simulink subsystem "FlexibleDriveline"  (R2025b)
settings: Solver=VariableStepAuto  StartTime=0.0  StopTime=10.0  RelTol=1e-3
PreLoadFcn:
  | FlexibleDrivelineParams;
undefined symbols (not defined in the file or in its folder): flexDLParams, fs
libraries: fl_lib x41, sdl_lib x24, nesl_utility x3
(part 1 of 2)
settings Model: Creator=shachind  LastModifiedBy=shachind

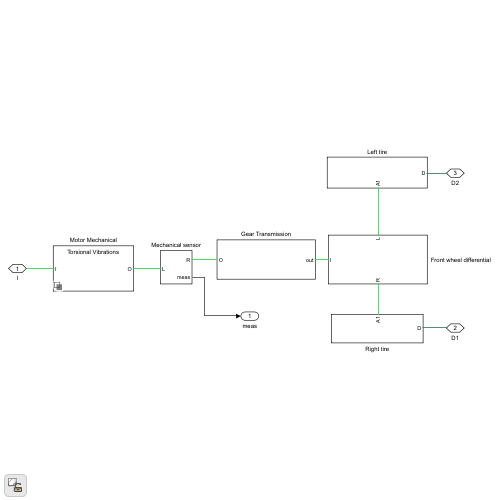
[thumbnail: Simulink's stored preview of the top-level diagram]
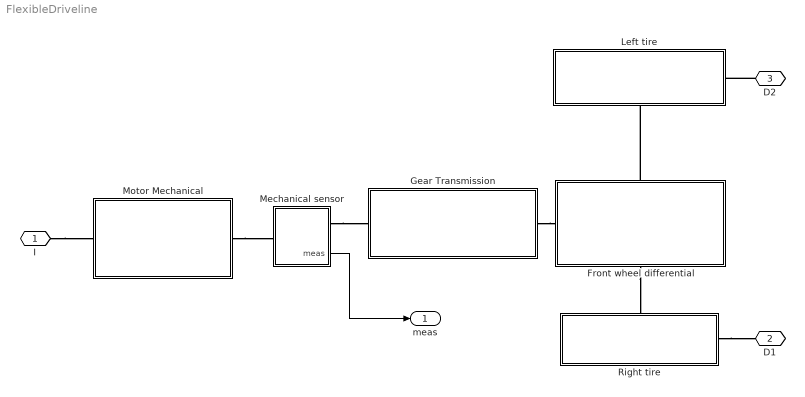
== system FlexibleDriveline ==
  Front wheel differential : Subsystem
      settings: PortSchema="{\"entries\":[{\"content\":{\"sides\":[{\"content\":{\"connectorIds\":[\"LConn1\"]},\"type\":\"ConnectorPlacement.EquallySpacedRectSide\",\"uuid\":\"c11434d0-9930-428a-bdcc-d2cb24030201\"},{\"content\":{\"connectorIds\":[\"RConn1\"],\"side\":\"RIGHT\"},\"type\":\"ConnectorPlacement.EquallySpacedRectSide\",\"uuid\":\"94e78a84-1cc1-4194-8e32-79b35f643a00\"},{\"content\":{\"side\":\"TOP\"},\"type\":\"ConnectorPlacement.EquallySpacedRectSide\",\"uuid\":\"2a2ff05c-1e68-4433-96e8-1c1d7698d135\"},{\"content\":{\"connectorIds\":[\"RConn2\"],\"side\":\"BOTTOM\"},\"type\":\"ConnectorPlacement.EquallySpacedRectSide\",\"uuid\":\"79f74731-f04d-4ec7-8450-045a74f69ecc\"}]},\"type\":\"ConnectorPlacement.EquallySpacedConnector\",\"uuid\":\"ade08aca-446e-4c23-b476-7b46661d2103\"}],\"packageUris\":[\"http://schema.mathworks.com/mf0/Connector/R2020b\"],\"version\":\"1.0\"}"
  Gear Transmission : Subsystem
  Left tire : Subsystem
      settings: PortSchema="{\"entries\":[{\"content\":{\"sides\":[{\"content\":{},\"type\":\"ConnectorPlacement.EquallySpacedRectSide\",\"uuid\":\"a6e63744-e74e-4c59-9a73-9f5bb4c6dc5e\"},{\"content\":{\"connectorIds\":[\"RConn1\"],\"side\":\"RIGHT\"},\"type\":\"ConnectorPlacement.EquallySpacedRectSide\",\"uuid\":\"cd80d7a6-bc64-46ff-87eb-327b10d625d4\"},{\"content\":{\"side\":\"TOP\"},\"type\":\"ConnectorPlacement.EquallySpacedRectSide\",\"uuid\":\"654a6e45-7395-4805-a08f-34f7a106fd1a\"},{\"content\":{\"connectorIds\":[\"RConn2\"],\"side\":\"BOTTOM\"},\"type\":\"ConnectorPlacement.EquallySpacedRectSide\",\"uuid\":\"572e738d-5229-4313-b0e3-7599b587bb85\"}]},\"type\":\"ConnectorPlacement.EquallySpacedConnector\",\"uuid\":\"3d8eeb69-cd59-4894-aa80-d96e9faae830\"}],\"packageUris\":[\"http://schema.mathworks.com/mf0/Connector/R2020b\"],\"version\":\"1.0\"}"
  Mechanical sensor : Subsystem
      settings: PortSchema="{\"entries\":[{\"content\":{\"sides\":[{\"content\":{\"connectorIds\":[\"LConn1\",\"Out1\"]},\"type\":\"ConnectorPlacement.EquallySpacedRectSide\",\"uuid\":\"9d0b7eaf-5dbc-4711-a9f9-5254d5ad2438\"},{\"content\":{\"connectorIds\":[\"RConn1\"],\"side\":\"RIGHT\"},\"type\":\"ConnectorPlacement.EquallySpacedRectSide\",\"uuid\":\"1084bd7e-accf-404d-815d-6b48331d5fd1\"},{\"content\":{\"side\":\"TOP\"},\"type\":\"ConnectorPlacement.EquallySpacedRectSide\",\"uuid\":\"4e1c109f-5704-45c2-8a88-7bde344122da\"}]},\"type\":\"ConnectorPlacement.EquallySpacedConnector\",\"uuid\":\"e6b98985-8de9-437e-9e9a-976cda41402d\"}],\"packageUris\":[\"http://schema.mathworks.com/mf0/Connector/R2020b\"],\"version\":\"1.0\"}"
  Motor Mechanical : Subsystem  Variant=on  VariantControlMode=label  LabelModeActiveChoice=true
  Right tire : Subsystem
      settings: PortSchema="{\"entries\":[{\"content\":{\"sides\":[{\"content\":{\"connectorIds\":[\"LConn1\"]},\"type\":\"ConnectorPlacement.EquallySpacedRectSide\",\"uuid\":\"a6e63744-e74e-4c59-9a73-9f5bb4c6dc5e\"},{\"content\":{\"side\":\"RIGHT\"},\"type\":\"ConnectorPlacement.EquallySpacedRectSide\",\"uuid\":\"cd80d7a6-bc64-46ff-87eb-327b10d625d4\"},{\"content\":{\"side\":\"TOP\"},\"type\":\"ConnectorPlacement.EquallySpacedRectSide\",\"uuid\":\"654a6e45-7395-4805-a08f-34f7a106fd1a\"},{\"content\":{\"connectorIds\":[\"RConn1\"],\"side\":\"BOTTOM\"},\"type\":\"ConnectorPlacement.EquallySpacedRectSide\",\"uuid\":\"572e738d-5229-4313-b0e3-7599b587bb85\"}]},\"type\":\"ConnectorPlacement.EquallySpacedConnector\",\"uuid\":\"3d8eeb69-cd59-4894-aa80-d96e9faae830\"}],\"packageUris\":[\"http://schema.mathworks.com/mf0/Connector/R2020b\"],\"version\":\"1.0\"}"
  I : PMIOPort  Side=Left
  D1 : PMIOPort  Port=2  Side=Right
  D2 : PMIOPort  Port=3  Side=Right
  meas : Outport
  wires:
  Mechanical sensor/1(meas) -> meas/1
  connections:
  Front wheel differential/RConn1 -- Right tire/RConn1
  Front wheel differential/LConn1 -- Left tire/RConn2
  Right tire/LConn1 -- D1/RConn1
  Gear Transmission/LConn1 -- Front wheel differential/RConn2
  D2/RConn1 -- Left tire/RConn1
  I/RConn1 -- Motor Mechanical/LConn1
  Mechanical sensor/LConn1 -- Gear Transmission/RConn1
  Motor Mechanical/RConn1 -- Mechanical sensor/RConn1

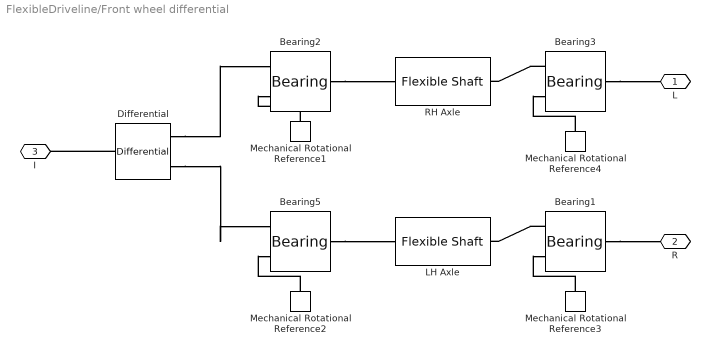
== system FlexibleDriveline/Front wheel differential ==
  Bearing{1..3,5} (4 alike) : sdl_lib/Couplings & Drives/Bearing  bearingType=sdl.enum.bearingType.BallRoller  enableFollower=true  casing=true  radius=30 mm  length=100 mm  loadType=foundation.enum.constant_variable.constant  load=10 N  F_thr=0.001 N  w_thr=0.001 rev/s  frictionType=foundation.enum.constant_variable.constant  interp_method_1=simscape.enum.interpolation.linear  extrap_method_1=simscape.enum.extrapolation.linear  f_coeff=0.002  N_TLU=[10, 2500, 5000, 10000, 25000] rpm  f_coeff_TLU=[.004, .001, .0005, .00025, .000125]  customizeFrictionCurve=false  mu=0.29 Pa*s  visc_coeff_min=0.002  bearingModulus=7.2519e-08 rev  muN_P_norm_TLU=[.4306, .6124, .6651, .7512, .866, 1, 1.1962, 1.4354, 3.8517]  visc_coeff_norm_TLU=[3.6621, 1.672, 1.3397, 1.1811, 1.0743, 1, 1.0358, 1.1173, 2.2792]  interp_method_2=simscape.enum.interpolation.linear  extrap_method_2=simscape.enum.extrapolation.linear
      settings: InternalSimscapePortConfiguration="{\"Bottom\":[{\"id\":\"C\",\"label\":\"C\",\"type\":\"foundation.mechanical.rotational.rotational\"}],\"Left\":[{\"id\":\"B\",\"label\":\"B\",\"type\":\"foundation.mechanical.rotational.rotational\"}],\"Right\":[{\"id\":\"F\",\"label\":\"F\",\"type\":\"foundation.mechanical.rotational.rotational\"}],\"Top\":[]}"
  Differential : sdl_lib/Gears/Differential  driveshaft_location=sdl.enum.differential_orientation.right  cd_ratio=finalDriveGearRatio  friction_model=sdl.enum.gear_friction.constant  efficiency=flexDLParams.gearBox.sunAndCarrierEfficiency  temperature_TLU=[280, 300, 320] K  efficiency_ss_TLU=[.95, .9, .85]  efficiency_cd_TLU=[.95, .9, .85]  pwr_thr=[.001, .001] W  mu_visc=[0, 0] N*m*s/rad  model_inertia=true  sun_inertia=0.001 kg*m^2  sun_radius=0.0001 m  carrier_inertia=flexDLParams.gearBox.finalGearInertia kg*m^2  planet_inertia=0.001 kg*m^2  planet_mass=0.001 kg  thermal_mass=50 J/K  T_init=300 K
  LH Axle : sdl_lib/Couplings & Drives/Flexible Shaft  modelTorsion=true  modelTransverse=false  n_segments=1  parameterization=sdl.enum.shaftParameterization.MaterialProperties  length=1 m  lengths=[1, .5, .25] m  shaft_stiffness=2e5 N*m/rad  shaft_inertia=0.02 kg*m^2  shaft_stiffnesses=[400000, 200000, 100000] N*m/rad  shaft_inertias=[.025, .02, .015] kg*m^2  eiIN=5e5 Pa*m^4  rhoaIN=19 kg/m  eiINs=[600000, 500000, 400000] Pa*m^4  rhoaINs=[20, 19, 18] kg/m  density=7.8e3 kg/m^3  shear_modulus=7.93e9 Pa  elastic_modulus=200e9 Pa  shaft_construction=sdl.enum.shaftConstruction.solid  diameter_outer=0.075 m  diameter_inner=0.05 m  diameter_outers=[.085, .075, .065] m  diameter_inners=[.055, .05, .045] m  damping_ratio=0.01  mu_visc_BF=[0, 0] N*m*s/rad  mu_visc=[0, 0] N*m*s/rad  initial_deflection=0 rad  initial_velocity=0 rpm  num_supports=sdl.enum.num_supports.two  z_support=[0, 0.5] m  boundaryB1=sdl.enum.shaftSupport.clamp  DrotB1_row=[1000, 1000] N*m*s/rad  DtransB1_row=[20000, -44000, -44000, 350000] N*s/m  DtransB1_w_mat=[20000, -44000, -44000, 350000; 10000, -25000, -25000, 140000; 5000, -10000, -10000, 20000] N*s/m  KrotB1_row=[10000, 10000] N*m/rad  KtransB1_row=[1000000, -200000, -300000, 5000000] N/m  KtransB1_w_mat=[1000000, -600000, -3500000, 8000000; 1000000, -200000, -3000000, 5000000; 1000000, -50000, -2500000, 3000000] N/m  boundaryI1=sdl.enum.shaftSupport.clamp  DrotI1_row=[1000, 1000] N*m*s/rad  DtransI1_row=[20000, -44000, -44000, 350000] N*s/m  DtransI1_w_mat=[20000, -44000, -44000, 350000; 10000, -25000, -25000, 140000; 5000, -10000, -10000, 20000] N*s/m  KrotI1_row=[10000, 10000] N*m/rad  KtransI1_row=[1000000, -200000, -300000, 5000000] N/m  KtransI1_w_mat=[1000000, -600000, -3500000, 8000000; 1000000, -200000, -3000000, 5000000; 1000000, -50000, -2500000, 3000000] N/m  boundaryI2=sdl.enum.shaftSupport.clamp  DrotI2_row=[1000, 1000] N*m*s/rad  DtransI2_row=[20000, -44000, -44000, 350000] N*s/m  DtransI2_w_mat=[20000, -44000, -44000, 350000; 10000, -25000, -25000, 140000; 5000, -10000, -10000, 20000] N*s/m  KrotI2_row=[10000, 10000] N*m/rad  KtransI2_row=[1000000, -200000, -300000, 5000000] N/m  KtransI2_w_mat=[1000000, -600000, -3500000, 8000000; 1000000, -200000, -3000000, 5000000; 1000000, -50000, -2500000, 3000000] N/m  boundaryF1=sdl.enum.shaftSupport.clamp  DrotF1_row=[1000, 1000] N*m*s/rad  DtransF1_row=[20000, -44000, -44000, 350000] N*s/m  DtransF1_w_mat=[20000, -44000, -44000, 350000; 10000, -25000, -25000, 140000; 5000, -10000, -10000, 20000] N*s/m  KrotF1_row=[10000, 10000] N*m/rad  KtransF1_row=[1000000, -200000, -300000, 5000000] N/m  KtransF1_w_mat=[1000000, -600000, -3500000, 8000000; 1000000, -200000, -3000000, 5000000; 1000000, -50000, -2500000, 3000000] N/m  bearing_speed=[200, 500, 1500] rpm  alpha=10 1/s  beta=1e-8 s  noDisk=sdl.enum.shaftDisks.none  zDisk=0.5 m  mDiskIN=2 kg  IdDiskIN=0.025 kg*m^2  IpDiskIN=0.050 kg*m^2  enable_static_unbalance=true  offsetMR=[.01, .01] kg*m  offsetMR_initialAngleIN=[0, pi] rad  offsetMassLocation=[.33, .67] m  enable_external_force=false  externalForce=[1, 2] N  externalForceHarmonic=[.5, 2]  externalLoadAngle=[pi / 2, 3 * pi / 4] rad  zExternalLoad=[.25, .75] m  AnalysisMethod=sdl.enum.bendingAnalysisMethod.LumpedMass  ModeInputMethod=sdl.enum.modeInputMethod.SimscapeDetermined  numModesIn=6  mode_speed_dependency=sdl.enum.mode_speed_dependency.Static  OmegaNom=5000 rpm  wMax=1e8 rpm  dz=0.01 m  userMode_w=[280, 644, 615, 1285] rad/s  userMode_w_mat=[257, 780, 580, 1560; 280, 644, 615, 1285; 294, 513, 636, 1020] rad/s  userMode_z=[0, .1, .2, .3, .4, .5, .6, .7, .8, .9, 1] m  userMode_shapeX=[.1648, .0086, -.2759, .0162; .1671, .0093, -.2231, .0133; .1691, .01, -.1689, .0102; .1707, .0105, -.1135, .007; .1717, .0108, -.057, .0035; .1721, .0109, 0, 0; .1717, .0108, .057, -.0035; .1707, .0105, .1135, -.007; .1691, .01, .1689, -.0102; .1671, .0093, .2231, -.0133; .1648, .0086, .2759, -.0162]  userMode_shapeX_mat=cat(3, [.1842, .0134, -.3072, .0272; .1863, .0152, -.2482, .0226; .1882, .0169, -.1878, .0176; .1897, .0182, -.1261, .0121; .1906, .019, -.0634, .0062; .191, .0193, 0, 0; .1906, .019, .0634, -.0062; .1897, .0182, .1261, -.0121; .1882, .0169, .1878, -.0176; .1863, .0152, .2482, -.0226; .1842, .0134, .3072, -.0272], [.1648, .0086, -.2759, .0162; .1671, .0093, -.2231, .0133; .1691, .01, -.1689, .0102; .1707, .0105, -.1135, .007; .1717, .0108, -.057, .0035; .1721, .0109, 0, 0; .1717, .0108, .057, -.0035; .1707, .0105, .1135, -.007; .1691, .01, .1689, -.0102; .1671, .0093, .2231, -.0133; .1648, .0086, .2759, -.0162], [.1291, .0046, -.2166, .0082; .131, .0048, -.1751, .0067; .1327, .005, -.1327, .0051; .1341, .0052, -.0891, .0035; .135, .0053, -.0448, .0017; .1353, .0053, 0, 0; .135, .0053, .0448, -.0017; .1341, .0052, .0891, -.0035; .1327, .005, .1327, -.0051; .131, .0048, .1751, -.0067; .1291, .0046, .2166, -.0082])  userMode_shapeY=[.1193, -.1784, -.1997, -.3348; .1209, -.1933, -.1615, -.2751; .1224, -.2068, -.1223, -.2119; .1235, -.2176, -.0821, -.1445; .1243, -.2245, -.0413, -.0734; .1246, -.2269, 0, 0; .1243, -.2245, .0413, .0734; .1235, -.2176, .0821, .1445; .1224, -.2068, .1223, .2119; .1209, -.1933, .1615, .2751; .1193, -.1784, .1997, .3348]  userMode_shapeY_mat=cat(3, [.0885, -.1625, -.1475, -.3301; .0895, -.1847, -.1192, -.2745; .0904, -.2048, -.0902, -.2141; .0911, -.2209, -.0606, -.1475; .0916, -.2313, -.0304, -.0754; .0917, -.2349, 0, 0; .0916, -.2313, .0304, .0754; .0911, -.2209, .0606, .1475; .0904, -.2048, .0902, .2141; .0895, -.1847, .1192, .2745; .0885, -.1625, .1475, .3301], [.1193, -.1784, -.1997, -.3348; .1209, -.1933, -.1615, -.2751; .1224, -.2068, -.1223, -.2119; .1235, -.2176, -.0821, -.1445; .1243, -.2245, -.0413, -.0734; .1246, -.2269, 0, 0; .1243, -.2245, .0413, .0734; .1235, -.2176, .0821, .1445; .1224, -.2068, .1223, .2119; .1209, -.1933, .1615, .2751; .1193, -.1784, .1997, .3348], [.1566, -.1901, -.2628, -.3377; .1589, -.1994, -.2125, -.2753; .161, -.2079, -.1609, -.2103; .1627, -.2146, -.1081, -.1424; .1638, -.219, -.0544, -.0719; .1642, -.2205, 0, 0; .1638, -.219, .0544, .0719; .1627, -.2146, .1081, .1424; .161, -.2079, .1609, .2103; .1589, -.1994, .2125, .2753; .1566, -.1901, .2628, .3377])  eta_lumped_nominal=1  etaDer_lumped_nominal=1  eta_modal_nominal=1  etaDer_modal_nominal=1
      settings: InternalSimscapePortConfiguration="{\"Bottom\":[],\"Left\":[{\"id\":\"B\",\"label\":\"B\",\"type\":\"foundation.mechanical.rotational.rotational\"}],\"Right\":[{\"id\":\"F\",\"label\":\"F\",\"type\":\"foundation.mechanical.rotational.rotational\"}],\"Top\":[]}"
  Mechanical Rotational Reference{1..4} (4 alike) : fl_lib/Mechanical/Rotational Elements/Mechanical Rotational Reference
  RH Axle : sdl_lib/Couplings & Drives/Flexible Shaft  modelTorsion=true  modelTransverse=false  n_segments=1  parameterization=sdl.enum.shaftParameterization.MaterialProperties  length=0.5 m  lengths=[1, .5, .25] m  shaft_stiffness=1e5 N*m/rad  shaft_inertia=0.02 kg*m^2  shaft_stiffnesses=[400000, 200000, 100000] N*m/rad  shaft_inertias=[.025, .02, .015] kg*m^2  eiIN=5e5 Pa*m^4  rhoaIN=19 kg/m  eiINs=[600000, 500000, 400000] Pa*m^4  rhoaINs=[20, 19, 18] kg/m  density=7.8e3 kg/m^3  shear_modulus=7.93e9 Pa  elastic_modulus=200e9 Pa  shaft_construction=sdl.enum.shaftConstruction.solid  diameter_outer=0.075 m  diameter_inner=0.05 m  diameter_outers=[.085, .075, .065] m  diameter_inners=[.055, .05, .045] m  damping_ratio=0.01  mu_visc_BF=[0, 0] N*m*s/rad  mu_visc=[0, 0] N*m*s/rad  initial_deflection=0 rad  initial_velocity=0 rpm  num_supports=sdl.enum.num_supports.two  z_support=[0, 0.5] m  boundaryB1=sdl.enum.shaftSupport.clamp  DrotB1_row=[1000, 1000] N*m*s/rad  DtransB1_row=[20000, -44000, -44000, 350000] N*s/m  DtransB1_w_mat=[20000, -44000, -44000, 350000; 10000, -25000, -25000, 140000; 5000, -10000, -10000, 20000] N*s/m  KrotB1_row=[10000, 10000] N*m/rad  KtransB1_row=[1000000, -200000, -300000, 5000000] N/m  KtransB1_w_mat=[1000000, -600000, -3500000, 8000000; 1000000, -200000, -3000000, 5000000; 1000000, -50000, -2500000, 3000000] N/m  boundaryI1=sdl.enum.shaftSupport.clamp  DrotI1_row=[1000, 1000] N*m*s/rad  DtransI1_row=[20000, -44000, -44000, 350000] N*s/m  DtransI1_w_mat=[20000, -44000, -44000, 350000; 10000, -25000, -25000, 140000; 5000, -10000, -10000, 20000] N*s/m  KrotI1_row=[10000, 10000] N*m/rad  KtransI1_row=[1000000, -200000, -300000, 5000000] N/m  KtransI1_w_mat=[1000000, -600000, -3500000, 8000000; 1000000, -200000, -3000000, 5000000; 1000000, -50000, -2500000, 3000000] N/m  boundaryI2=sdl.enum.shaftSupport.clamp  DrotI2_row=[1000, 1000] N*m*s/rad  DtransI2_row=[20000, -44000, -44000, 350000] N*s/m  DtransI2_w_mat=[20000, -44000, -44000, 350000; 10000, -25000, -25000, 140000; 5000, -10000, -10000, 20000] N*s/m  KrotI2_row=[10000, 10000] N*m/rad  KtransI2_row=[1000000, -200000, -300000, 5000000] N/m  KtransI2_w_mat=[1000000, -600000, -3500000, 8000000; 1000000, -200000, -3000000, 5000000; 1000000, -50000, -2500000, 3000000] N/m  boundaryF1=sdl.enum.shaftSupport.clamp  DrotF1_row=[1000, 1000] N*m*s/rad  DtransF1_row=[20000, -44000, -44000, 350000] N*s/m  DtransF1_w_mat=[20000, -44000, -44000, 350000; 10000, -25000, -25000, 140000; 5000, -10000, -10000, 20000] N*s/m  KrotF1_row=[10000, 10000] N*m/rad  KtransF1_row=[1000000, -200000, -300000, 5000000] N/m  KtransF1_w_mat=[1000000, -600000, -3500000, 8000000; 1000000, -200000, -3000000, 5000000; 1000000, -50000, -2500000, 3000000] N/m  bearing_speed=[200, 500, 1500] rpm  alpha=10 1/s  beta=1e-8 s  noDisk=sdl.enum.shaftDisks.none  zDisk=0.5 m  mDiskIN=2 kg  IdDiskIN=0.025 kg*m^2  IpDiskIN=0.050 kg*m^2  enable_static_unbalance=true  offsetMR=[.01, .01] kg*m  offsetMR_initialAngleIN=[0, pi] rad  offsetMassLocation=[.33, .67] m  enable_external_force=false  externalForce=[1, 2] N  externalForceHarmonic=[.5, 2]  externalLoadAngle=[pi / 2, 3 * pi / 4] rad  zExternalLoad=[.25, .75] m  AnalysisMethod=sdl.enum.bendingAnalysisMethod.LumpedMass  ModeInputMethod=sdl.enum.modeInputMethod.SimscapeDetermined  numModesIn=6  mode_speed_dependency=sdl.enum.mode_speed_dependency.Static  OmegaNom=5000 rpm  wMax=1e8 rpm  dz=0.01 m  userMode_w=[280, 644, 615, 1285] rad/s  userMode_w_mat=[257, 780, 580, 1560; 280, 644, 615, 1285; 294, 513, 636, 1020] rad/s  userMode_z=[0, .1, .2, .3, .4, .5, .6, .7, .8, .9, 1] m  userMode_shapeX=[.1648, .0086, -.2759, .0162; .1671, .0093, -.2231, .0133; .1691, .01, -.1689, .0102; .1707, .0105, -.1135, .007; .1717, .0108, -.057, .0035; .1721, .0109, 0, 0; .1717, .0108, .057, -.0035; .1707, .0105, .1135, -.007; .1691, .01, .1689, -.0102; .1671, .0093, .2231, -.0133; .1648, .0086, .2759, -.0162]  userMode_shapeX_mat=cat(3, [.1842, .0134, -.3072, .0272; .1863, .0152, -.2482, .0226; .1882, .0169, -.1878, .0176; .1897, .0182, -.1261, .0121; .1906, .019, -.0634, .0062; .191, .0193, 0, 0; .1906, .019, .0634, -.0062; .1897, .0182, .1261, -.0121; .1882, .0169, .1878, -.0176; .1863, .0152, .2482, -.0226; .1842, .0134, .3072, -.0272], [.1648, .0086, -.2759, .0162; .1671, .0093, -.2231, .0133; .1691, .01, -.1689, .0102; .1707, .0105, -.1135, .007; .1717, .0108, -.057, .0035; .1721, .0109, 0, 0; .1717, .0108, .057, -.0035; .1707, .0105, .1135, -.007; .1691, .01, .1689, -.0102; .1671, .0093, .2231, -.0133; .1648, .0086, .2759, -.0162], [.1291, .0046, -.2166, .0082; .131, .0048, -.1751, .0067; .1327, .005, -.1327, .0051; .1341, .0052, -.0891, .0035; .135, .0053, -.0448, .0017; .1353, .0053, 0, 0; .135, .0053, .0448, -.0017; .1341, .0052, .0891, -.0035; .1327, .005, .1327, -.0051; .131, .0048, .1751, -.0067; .1291, .0046, .2166, -.0082])  userMode_shapeY=[.1193, -.1784, -.1997, -.3348; .1209, -.1933, -.1615, -.2751; .1224, -.2068, -.1223, -.2119; .1235, -.2176, -.0821, -.1445; .1243, -.2245, -.0413, -.0734; .1246, -.2269, 0, 0; .1243, -.2245, .0413, .0734; .1235, -.2176, .0821, .1445; .1224, -.2068, .1223, .2119; .1209, -.1933, .1615, .2751; .1193, -.1784, .1997, .3348]  userMode_shapeY_mat=cat(3, [.0885, -.1625, -.1475, -.3301; .0895, -.1847, -.1192, -.2745; .0904, -.2048, -.0902, -.2141; .0911, -.2209, -.0606, -.1475; .0916, -.2313, -.0304, -.0754; .0917, -.2349, 0, 0; .0916, -.2313, .0304, .0754; .0911, -.2209, .0606, .1475; .0904, -.2048, .0902, .2141; .0895, -.1847, .1192, .2745; .0885, -.1625, .1475, .3301], [.1193, -.1784, -.1997, -.3348; .1209, -.1933, -.1615, -.2751; .1224, -.2068, -.1223, -.2119; .1235, -.2176, -.0821, -.1445; .1243, -.2245, -.0413, -.0734; .1246, -.2269, 0, 0; .1243, -.2245, .0413, .0734; .1235, -.2176, .0821, .1445; .1224, -.2068, .1223, .2119; .1209, -.1933, .1615, .2751; .1193, -.1784, .1997, .3348], [.1566, -.1901, -.2628, -.3377; .1589, -.1994, -.2125, -.2753; .161, -.2079, -.1609, -.2103; .1627, -.2146, -.1081, -.1424; .1638, -.219, -.0544, -.0719; .1642, -.2205, 0, 0; .1638, -.219, .0544, .0719; .1627, -.2146, .1081, .1424; .161, -.2079, .1609, .2103; .1589, -.1994, .2125, .2753; .1566, -.1901, .2628, .3377])  eta_lumped_nominal=1  etaDer_lumped_nominal=1  eta_modal_nominal=1  etaDer_modal_nominal=1
      settings: InternalSimscapePortConfiguration="{\"Bottom\":[],\"Left\":[{\"id\":\"B\",\"label\":\"B\",\"type\":\"foundation.mechanical.rotational.rotational\"}],\"Right\":[{\"id\":\"F\",\"label\":\"F\",\"type\":\"foundation.mechanical.rotational.rotational\"}],\"Top\":[]}"
  L : PMIOPort  Side=Left
  R : PMIOPort  Port=2  Side=Right
  I : PMIOPort  Port=3  Side=Right
  connections:
  Mechanical Rotational Reference4/LConn1 -- Bearing3/RConn2
  Bearing3/LConn1 -- L/RConn1
  Bearing3/RConn1 -- RH Axle/RConn1
  Mechanical Rotational Reference3/LConn1 -- Bearing1/RConn2
  Bearing1/RConn1 -- LH Axle/RConn1
  Bearing1/LConn1 -- R/RConn1
  Mechanical Rotational Reference2/LConn1 -- Bearing5/RConn2
  Mechanical Rotational Reference1/LConn1 -- Bearing2/RConn2
  Differential/LConn1 -- I/RConn1
  Bearing2/LConn1 -- RH Axle/LConn1
  Bearing5/LConn1 -- LH Axle/LConn1
  Differential/RConn2 -- Bearing2/RConn1
  Differential/RConn1 -- Bearing5/RConn1

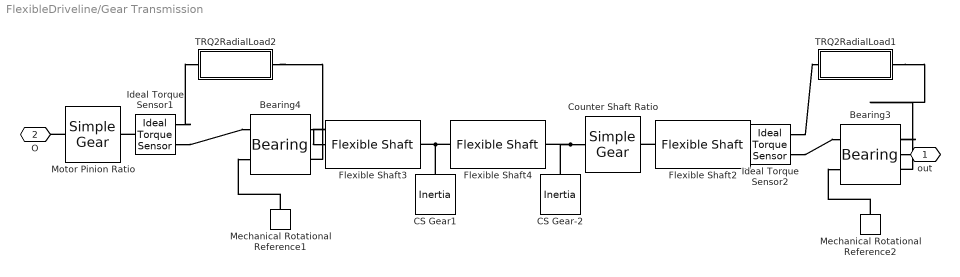
== system FlexibleDriveline/Gear Transmission ==
  Bearing3 : sdl_lib/Couplings & Drives/Bearing  bearingType=sdl.enum.bearingType.BallRoller  enableFollower=true  casing=true  radius=30 mm  length=100 mm  loadType=foundation.enum.constant_variable.variable  load=10 N  F_thr=0.001 N  w_thr=0.001 rev/s  frictionType=foundation.enum.constant_variable.constant  interp_method_1=simscape.enum.interpolation.linear  extrap_method_1=simscape.enum.extrapolation.linear  f_coeff=0.002  N_TLU=[10, 2500, 5000, 10000, 25000] rpm  f_coeff_TLU=[.004, .001, .0005, .00025, .000125]  customizeFrictionCurve=false  mu=0.29 Pa*s  visc_coeff_min=0.002  bearingModulus=7.2519e-08 rev  muN_P_norm_TLU=[.4306, .6124, .6651, .7512, .866, 1, 1.1962, 1.4354, 3.8517]  visc_coeff_norm_TLU=[3.6621, 1.672, 1.3397, 1.1811, 1.0743, 1, 1.0358, 1.1173, 2.2792]  interp_method_2=simscape.enum.interpolation.linear  extrap_method_2=simscape.enum.extrapolation.linear
      settings: InternalSimscapePortConfiguration="{\"Bottom\":[{\"id\":\"C\",\"label\":\"C\",\"type\":\"foundation.mechanical.rotational.rotational\"}],\"Left\":[{\"id\":\"B\",\"label\":\"B\",\"type\":\"foundation.mechanical.rotational.rotational\"}],\"Right\":[{\"id\":\"F\",\"label\":\"F\",\"type\":\"foundation.mechanical.rotational.rotational\"}],\"Top\":[{\"id\":\"Force\",\"label\":\"Load\",\"type\":\"input\"}]}"
  Bearing4 : sdl_lib/Couplings & Drives/Bearing  bearingType=sdl.enum.bearingType.BallRoller  enableFollower=true  casing=true  radius=30 mm  length=100 mm  loadType=foundation.enum.constant_variable.variable  load=10 N  F_thr=0.001 N  w_thr=0.001 rev/s  frictionType=foundation.enum.constant_variable.constant  interp_method_1=simscape.enum.interpolation.linear  extrap_method_1=simscape.enum.extrapolation.linear  f_coeff=0.002  N_TLU=[10, 2500, 5000, 10000, 25000] rpm  f_coeff_TLU=[.004, .001, .0005, .00025, .000125]  customizeFrictionCurve=false  mu=0.29 Pa*s  visc_coeff_min=0.002  bearingModulus=7.2519e-08 rev  muN_P_norm_TLU=[.4306, .6124, .6651, .7512, .866, 1, 1.1962, 1.4354, 3.8517]  visc_coeff_norm_TLU=[3.6621, 1.672, 1.3397, 1.1811, 1.0743, 1, 1.0358, 1.1173, 2.2792]  interp_method_2=simscape.enum.interpolation.linear  extrap_method_2=simscape.enum.extrapolation.linear
      settings: InternalSimscapePortConfiguration="{\"Bottom\":[{\"id\":\"C\",\"label\":\"C\",\"type\":\"foundation.mechanical.rotational.rotational\"}],\"Left\":[{\"id\":\"B\",\"label\":\"B\",\"type\":\"foundation.mechanical.rotational.rotational\"}],\"Right\":[{\"id\":\"F\",\"label\":\"F\",\"type\":\"foundation.mechanical.rotational.rotational\"}],\"Top\":[{\"id\":\"Force\",\"label\":\"Load\",\"type\":\"input\"}]}"
  CS Gear-2 : fl_lib/Mechanical/Rotational Elements/Inertia  inertia=flexDLParams.gearBox.gear2Inertia kg*m^2  num_ports=foundation.enum.numPorts2.one  w_specify=on  w_priority=High  w=0 rpm  w_nominal_specify=off  w_nominal_value=1  w_nominal_unit=rad/s  t_specify=off  t_priority=High  t=0 N*m  t_nominal_specify=off  t_nominal_value=1  t_nominal_unit=N*m
  CS Gear1 : fl_lib/Mechanical/Rotational Elements/Inertia  inertia=flexDLParams.gearBox.gear1Inertia kg*m^2  num_ports=foundation.enum.numPorts2.one  w_specify=on  w_priority=High  w=0 rpm  w_nominal_specify=off  w_nominal_value=1  w_nominal_unit=rad/s  t_specify=off  t_priority=High  t=0 N*m  t_nominal_specify=off  t_nominal_value=1  t_nominal_unit=N*m
  Counter Shaft Ratio : sdl_lib/Gears/Simple Gear  ratio=CSToMSGearRatio  rotation_direction=sdl.enum.shaftOutputDirection.opposite  friction_model=sdl.enum.gear_efficiencies_load.off  T_noload=0.1 N*m  T_nom=5 N*m  efficiency_nom=0.8  efficiency=0.8  temperature_TLU=[280, 300, 320] K  load_TLU=[1, 5, 10] N*m  efficiency_TLU=[.95, .9, .85]  efficiency_TLU2=[.85, .8, .75; .95, .9, .85; .85, .8, .7]  w_thr=0.01 rad/s  pwr_thr=0.001 W  enable_backlash=true  hardstop_model=simscape.enum.hardstop.smooth  backlash_distance=flexDLParams.gearBox.gear2BackLash mm  r_base=flexDLParams.gearBox.gear2BaseRadius m  transition=1e-4 mm  backlash_stiffness=flexDLParams.gearBox.gear2Stiffness N/m  backlash_damping=flexDLParams.gearBox.gear2Damping N*s/m  coeff_rest=0.7  v_tol=0.001 m/s  f_tol=0.001 N  mu_visc=flexDLParams.gearBox.gear1ViscousDampingCoefficients N*m*s/rad  thermal_mass=50 J/K  temperature_specify=off  temperature_priority=High  temperature=300 K  temperature_nominal_specify=off  temperature_nominal_value=1  temperature_nominal_unit=K  x_backlash_specify=off  x_backlash_priority=None  x_backlash=0 mm  x_backlash_nominal_specify=off  x_backlash_nominal_value=1  x_backlash_nominal_unit=mm  f_hardstop_specify=off  f_hardstop_priority=None  f_hardstop=0 N  f_hardstop_nominal_specify=off  f_hardstop_nominal_value=1  f_hardstop_nominal_unit=N  v_backlash_specify=off  v_backlash_priority=None  v_backlash=0 m/s  v_backlash_nominal_specify=off  v_backlash_nominal_value=1  v_backlash_nominal_unit=m/s
  Flexible Shaft2 : sdl_lib/Couplings & Drives/Flexible Shaft  modelTorsion=true  modelTransverse=false  n_segments=1  parameterization=sdl.enum.shaftParameterization.StiffnessInertia  length=1 m  lengths=[1, .5, .25] m  shaft_stiffness=2e5 N*m/rad  shaft_inertia=0.02 kg*m^2  shaft_stiffnesses=[400000, 200000, 100000] N*m/rad  shaft_inertias=[.025, .02, .015] kg*m^2  eiIN=5e5 Pa*m^4  rhoaIN=19 kg/m  eiINs=[600000, 500000, 400000] Pa*m^4  rhoaINs=[20, 19, 18] kg/m  density=7.8e3 kg/m^3  shear_modulus=7.93e9 Pa  elastic_modulus=200e9 Pa  shaft_construction=sdl.enum.shaftConstruction.solid  diameter_outer=0.075 m  diameter_inner=0.05 m  diameter_outers=[.085, .075, .065] m  diameter_inners=[.055, .05, .045] m  damping_ratio=0.01  mu_visc_BF=[0, 0] N*m*s/rad  mu_visc=[0, 0] N*m*s/rad  initial_deflection=0 rad  initial_velocity=0 rpm  num_supports=sdl.enum.num_supports.two  z_support=[0, 1] m  boundaryB1=sdl.enum.shaftSupport.clamp  DrotB1_row=[1000, 1000] N*m*s/rad  DtransB1_row=[20000, -44000, -44000, 350000] N*s/m  DtransB1_w_mat=[20000, -44000, -44000, 350000; 10000, -25000, -25000, 140000; 5000, -10000, -10000, 20000] N*s/m  KrotB1_row=[10000, 10000] N*m/rad  KtransB1_row=[1000000, -200000, -300000, 5000000] N/m  KtransB1_w_mat=[1000000, -600000, -3500000, 8000000; 1000000, -200000, -3000000, 5000000; 1000000, -50000, -2500000, 3000000] N/m  boundaryI1=sdl.enum.shaftSupport.clamp  DrotI1_row=[1000, 1000] N*m*s/rad  DtransI1_row=[20000, -44000, -44000, 350000] N*s/m  DtransI1_w_mat=[20000, -44000, -44000, 350000; 10000, -25000, -25000, 140000; 5000, -10000, -10000, 20000] N*s/m  KrotI1_row=[10000, 10000] N*m/rad  KtransI1_row=[1000000, -200000, -300000, 5000000] N/m  KtransI1_w_mat=[1000000, -600000, -3500000, 8000000; 1000000, -200000, -3000000, 5000000; 1000000, -50000, -2500000, 3000000] N/m  boundaryI2=sdl.enum.shaftSupport.clamp  DrotI2_row=[1000, 1000] N*m*s/rad  DtransI2_row=[20000, -44000, -44000, 350000] N*s/m  DtransI2_w_mat=[20000, -44000, -44000, 350000; 10000, -25000, -25000, 140000; 5000, -10000, -10000, 20000] N*s/m  KrotI2_row=[10000, 10000] N*m/rad  KtransI2_row=[1000000, -200000, -300000, 5000000] N/m  KtransI2_w_mat=[1000000, -600000, -3500000, 8000000; 1000000, -200000, -3000000, 5000000; 1000000, -50000, -2500000, 3000000] N/m  boundaryF1=sdl.enum.shaftSupport.clamp  DrotF1_row=[1000, 1000] N*m*s/rad  DtransF1_row=[20000, -44000, -44000, 350000] N*s/m  DtransF1_w_mat=[20000, -44000, -44000, 350000; 10000, -25000, -25000, 140000; 5000, -10000, -10000, 20000] N*s/m  KrotF1_row=[10000, 10000] N*m/rad  KtransF1_row=[1000000, -200000, -300000, 5000000] N/m  KtransF1_w_mat=[1000000, -600000, -3500000, 8000000; 1000000, -200000, -3000000, 5000000; 1000000, -50000, -2500000, 3000000] N/m  bearing_speed=[200, 500, 1500] rpm  alpha=10 1/s  beta=1e-8 s  noDisk=sdl.enum.shaftDisks.none  zDisk=0.5 m  mDiskIN=2 kg  IdDiskIN=0.025 kg*m^2  IpDiskIN=0.050 kg*m^2  enable_static_unbalance=true  offsetMR=[.01, .01] kg*m  offsetMR_initialAngleIN=[0, pi] rad  offsetMassLocation=[.33, .67] m  enable_external_force=false  externalForce=[1, 2] N  externalForceHarmonic=[.5, 2]  externalLoadAngle=[pi / 2, 3 * pi / 4] rad  zExternalLoad=[.25, .75] m  AnalysisMethod=sdl.enum.bendingAnalysisMethod.LumpedMass  ModeInputMethod=sdl.enum.modeInputMethod.SimscapeDetermined  numModesIn=6  mode_speed_dependency=sdl.enum.mode_speed_dependency.Static  OmegaNom=5000 rpm  wMax=1e8 rpm  dz=0.01 m  userMode_w=[280, 644, 615, 1285] rad/s  userMode_w_mat=[257, 780, 580, 1560; 280, 644, 615, 1285; 294, 513, 636, 1020] rad/s  userMode_z=[0, .1, .2, .3, .4, .5, .6, .7, .8, .9, 1] m  userMode_shapeX=[.1648, .0086, -.2759, .0162; .1671, .0093, -.2231, .0133; .1691, .01, -.1689, .0102; .1707, .0105, -.1135, .007; .1717, .0108, -.057, .0035; .1721, .0109, 0, 0; .1717, .0108, .057, -.0035; .1707, .0105, .1135, -.007; .1691, .01, .1689, -.0102; .1671, .0093, .2231, -.0133; .1648, .0086, .2759, -.0162]  userMode_shapeX_mat=cat(3, [.1842, .0134, -.3072, .0272; .1863, .0152, -.2482, .0226; .1882, .0169, -.1878, .0176; .1897, .0182, -.1261, .0121; .1906, .019, -.0634, .0062; .191, .0193, 0, 0; .1906, .019, .0634, -.0062; .1897, .0182, .1261, -.0121; .1882, .0169, .1878, -.0176; .1863, .0152, .2482, -.0226; .1842, .0134, .3072, -.0272], [.1648, .0086, -.2759, .0162; .1671, .0093, -.2231, .0133; .1691, .01, -.1689, .0102; .1707, .0105, -.1135, .007; .1717, .0108, -.057, .0035; .1721, .0109, 0, 0; .1717, .0108, .057, -.0035; .1707, .0105, .1135, -.007; .1691, .01, .1689, -.0102; .1671, .0093, .2231, -.0133; .1648, .0086, .2759, -.0162], [.1291, .0046, -.2166, .0082; .131, .0048, -.1751, .0067; .1327, .005, -.1327, .0051; .1341, .0052, -.0891, .0035; .135, .0053, -.0448, .0017; .1353, .0053, 0, 0; .135, .0053, .0448, -.0017; .1341, .0052, .0891, -.0035; .1327, .005, .1327, -.0051; .131, .0048, .1751, -.0067; .1291, .0046, .2166, -.0082])  userMode_shapeY=[.1193, -.1784, -.1997, -.3348; .1209, -.1933, -.1615, -.2751; .1224, -.2068, -.1223, -.2119; .1235, -.2176, -.0821, -.1445; .1243, -.2245, -.0413, -.0734; .1246, -.2269, 0, 0; .1243, -.2245, .0413, .0734; .1235, -.2176, .0821, .1445; .1224, -.2068, .1223, .2119; .1209, -.1933, .1615, .2751; .1193, -.1784, .1997, .3348]  userMode_shapeY_mat=cat(3, [.0885, -.1625, -.1475, -.3301; .0895, -.1847, -.1192, -.2745; .0904, -.2048, -.0902, -.2141; .0911, -.2209, -.0606, -.1475; .0916, -.2313, -.0304, -.0754; .0917, -.2349, 0, 0; .0916, -.2313, .0304, .0754; .0911, -.2209, .0606, .1475; .0904, -.2048, .0902, .2141; .0895, -.1847, .1192, .2745; .0885, -.1625, .1475, .3301], [.1193, -.1784, -.1997, -.3348; .1209, -.1933, -.1615, -.2751; .1224, -.2068, -.1223, -.2119; .1235, -.2176, -.0821, -.1445; .1243, -.2245, -.0413, -.0734; .1246, -.2269, 0, 0; .1243, -.2245, .0413, .0734; .1235, -.2176, .0821, .1445; .1224, -.2068, .1223, .2119; .1209, -.1933, .1615, .2751; .1193, -.1784, .1997, .3348], [.1566, -.1901, -.2628, -.3377; .1589, -.1994, -.2125, -.2753; .161, -.2079, -.1609, -.2103; .1627, -.2146, -.1081, -.1424; .1638, -.219, -.0544, -.0719; .1642, -.2205, 0, 0; .1638, -.219, .0544, .0719; .1627, -.2146, .1081, .1424; .161, -.2079, .1609, .2103; .1589, -.1994, .2125, .2753; .1566, -.1901, .2628, .3377])  eta_lumped_nominal=1  etaDer_lumped_nominal=1  eta_modal_nominal=1  etaDer_modal_nominal=1
      settings: InternalSimscapePortConfiguration="{\"Bottom\":[],\"Left\":[{\"id\":\"B\",\"label\":\"B\",\"type\":\"foundation.mechanical.rotational.rotational\"}],\"Right\":[{\"id\":\"F\",\"label\":\"F\",\"type\":\"foundation.mechanical.rotational.rotational\"}],\"Top\":[]}"
  Flexible Shaft3 : sdl_lib/Couplings & Drives/Flexible Shaft  modelTorsion=true  modelTransverse=false  n_segments=1  parameterization=sdl.enum.shaftParameterization.StiffnessInertia  length=1 m  lengths=[1, .5, .25] m  shaft_stiffness=2e5 N*m/rad  shaft_inertia=0.02 kg*m^2  shaft_stiffnesses=[400000, 200000, 100000] N*m/rad  shaft_inertias=[.025, .02, .015] kg*m^2  eiIN=5e5 Pa*m^4  rhoaIN=19 kg/m  eiINs=[600000, 500000, 400000] Pa*m^4  rhoaINs=[20, 19, 18] kg/m  density=7.8e3 kg/m^3  shear_modulus=7.93e9 Pa  elastic_modulus=200e9 Pa  shaft_construction=sdl.enum.shaftConstruction.solid  diameter_outer=0.075 m  diameter_inner=0.05 m  diameter_outers=[.085, .075, .065] m  diameter_inners=[.055, .05, .045] m  damping_ratio=0.01  mu_visc_BF=[0, 0] N*m*s/rad  mu_visc=[0, 0] N*m*s/rad  initial_deflection=0 rad  initial_velocity=0 rpm  num_supports=sdl.enum.num_supports.two  z_support=[0, 1] m  boundaryB1=sdl.enum.shaftSupport.clamp  DrotB1_row=[1000, 1000] N*m*s/rad  DtransB1_row=[20000, -44000, -44000, 350000] N*s/m  DtransB1_w_mat=[20000, -44000, -44000, 350000; 10000, -25000, -25000, 140000; 5000, -10000, -10000, 20000] N*s/m  KrotB1_row=[10000, 10000] N*m/rad  KtransB1_row=[1000000, -200000, -300000, 5000000] N/m  KtransB1_w_mat=[1000000, -600000, -3500000, 8000000; 1000000, -200000, -3000000, 5000000; 1000000, -50000, -2500000, 3000000] N/m  boundaryI1=sdl.enum.shaftSupport.clamp  DrotI1_row=[1000, 1000] N*m*s/rad  DtransI1_row=[20000, -44000, -44000, 350000] N*s/m  DtransI1_w_mat=[20000, -44000, -44000, 350000; 10000, -25000, -25000, 140000; 5000, -10000, -10000, 20000] N*s/m  KrotI1_row=[10000, 10000] N*m/rad  KtransI1_row=[1000000, -200000, -300000, 5000000] N/m  KtransI1_w_mat=[1000000, -600000, -3500000, 8000000; 1000000, -200000, -3000000, 5000000; 1000000, -50000, -2500000, 3000000] N/m  boundaryI2=sdl.enum.shaftSupport.clamp  DrotI2_row=[1000, 1000] N*m*s/rad  DtransI2_row=[20000, -44000, -44000, 350000] N*s/m  DtransI2_w_mat=[20000, -44000, -44000, 350000; 10000, -25000, -25000, 140000; 5000, -10000, -10000, 20000] N*s/m  KrotI2_row=[10000, 10000] N*m/rad  KtransI2_row=[1000000, -200000, -300000, 5000000] N/m  KtransI2_w_mat=[1000000, -600000, -3500000, 8000000; 1000000, -200000, -3000000, 5000000; 1000000, -50000, -2500000, 3000000] N/m  boundaryF1=sdl.enum.shaftSupport.clamp  DrotF1_row=[1000, 1000] N*m*s/rad  DtransF1_row=[20000, -44000, -44000, 350000] N*s/m  DtransF1_w_mat=[20000, -44000, -44000, 350000; 10000, -25000, -25000, 140000; 5000, -10000, -10000, 20000] N*s/m  KrotF1_row=[10000, 10000] N*m/rad  KtransF1_row=[1000000, -200000, -300000, 5000000] N/m  KtransF1_w_mat=[1000000, -600000, -3500000, 8000000; 1000000, -200000, -3000000, 5000000; 1000000, -50000, -2500000, 3000000] N/m  bearing_speed=[200, 500, 1500] rpm  alpha=10 1/s  beta=1e-8 s  noDisk=sdl.enum.shaftDisks.none  zDisk=0.5 m  mDiskIN=2 kg  IdDiskIN=0.025 kg*m^2  IpDiskIN=0.050 kg*m^2  enable_static_unbalance=true  offsetMR=[.01, .01] kg*m  offsetMR_initialAngleIN=[0, pi] rad  offsetMassLocation=[.33, .67] m  enable_external_force=false  externalForce=[1, 2] N  externalForceHarmonic=[.5, 2]  externalLoadAngle=[pi / 2, 3 * pi / 4] rad  zExternalLoad=[.25, .75] m  AnalysisMethod=sdl.enum.bendingAnalysisMethod.LumpedMass  ModeInputMethod=sdl.enum.modeInputMethod.SimscapeDetermined  numModesIn=6  mode_speed_dependency=sdl.enum.mode_speed_dependency.Static  OmegaNom=5000 rpm  wMax=1e8 rpm  dz=0.01 m  userMode_w=[280, 644, 615, 1285] rad/s  userMode_w_mat=[257, 780, 580, 1560; 280, 644, 615, 1285; 294, 513, 636, 1020] rad/s  userMode_z=[0, .1, .2, .3, .4, .5, .6, .7, .8, .9, 1] m  userMode_shapeX=[.1648, .0086, -.2759, .0162; .1671, .0093, -.2231, .0133; .1691, .01, -.1689, .0102; .1707, .0105, -.1135, .007; .1717, .0108, -.057, .0035; .1721, .0109, 0, 0; .1717, .0108, .057, -.0035; .1707, .0105, .1135, -.007; .1691, .01, .1689, -.0102; .1671, .0093, .2231, -.0133; .1648, .0086, .2759, -.0162]  userMode_shapeX_mat=cat(3, [.1842, .0134, -.3072, .0272; .1863, .0152, -.2482, .0226; .1882, .0169, -.1878, .0176; .1897, .0182, -.1261, .0121; .1906, .019, -.0634, .0062; .191, .0193, 0, 0; .1906, .019, .0634, -.0062; .1897, .0182, .1261, -.0121; .1882, .0169, .1878, -.0176; .1863, .0152, .2482, -.0226; .1842, .0134, .3072, -.0272], [.1648, .0086, -.2759, .0162; .1671, .0093, -.2231, .0133; .1691, .01, -.1689, .0102; .1707, .0105, -.1135, .007; .1717, .0108, -.057, .0035; .1721, .0109, 0, 0; .1717, .0108, .057, -.0035; .1707, .0105, .1135, -.007; .1691, .01, .1689, -.0102; .1671, .0093, .2231, -.0133; .1648, .0086, .2759, -.0162], [.1291, .0046, -.2166, .0082; .131, .0048, -.1751, .0067; .1327, .005, -.1327, .0051; .1341, .0052, -.0891, .0035; .135, .0053, -.0448, .0017; .1353, .0053, 0, 0; .135, .0053, .0448, -.0017; .1341, .0052, .0891, -.0035; .1327, .005, .1327, -.0051; .131, .0048, .1751, -.0067; .1291, .0046, .2166, -.0082])  userMode_shapeY=[.1193, -.1784, -.1997, -.3348; .1209, -.1933, -.1615, -.2751; .1224, -.2068, -.1223, -.2119; .1235, -.2176, -.0821, -.1445; .1243, -.2245, -.0413, -.0734; .1246, -.2269, 0, 0; .1243, -.2245, .0413, .0734; .1235, -.2176, .0821, .1445; .1224, -.2068, .1223, .2119; .1209, -.1933, .1615, .2751; .1193, -.1784, .1997, .3348]  userMode_shapeY_mat=cat(3, [.0885, -.1625, -.1475, -.3301; .0895, -.1847, -.1192, -.2745; .0904, -.2048, -.0902, -.2141; .0911, -.2209, -.0606, -.1475; .0916, -.2313, -.0304, -.0754; .0917, -.2349, 0, 0; .0916, -.2313, .0304, .0754; .0911, -.2209, .0606, .1475; .0904, -.2048, .0902, .2141; .0895, -.1847, .1192, .2745; .0885, -.1625, .1475, .3301], [.1193, -.1784, -.1997, -.3348; .1209, -.1933, -.1615, -.2751; .1224, -.2068, -.1223, -.2119; .1235, -.2176, -.0821, -.1445; .1243, -.2245, -.0413, -.0734; .1246, -.2269, 0, 0; .1243, -.2245, .0413, .0734; .1235, -.2176, .0821, .1445; .1224, -.2068, .1223, .2119; .1209, -.1933, .1615, .2751; .1193, -.1784, .1997, .3348], [.1566, -.1901, -.2628, -.3377; .1589, -.1994, -.2125, -.2753; .161, -.2079, -.1609, -.2103; .1627, -.2146, -.1081, -.1424; .1638, -.219, -.0544, -.0719; .1642, -.2205, 0, 0; .1638, -.219, .0544, .0719; .1627, -.2146, .1081, .1424; .161, -.2079, .1609, .2103; .1589, -.1994, .2125, .2753; .1566, -.1901, .2628, .3377])  eta_lumped_nominal=1  etaDer_lumped_nominal=1  eta_modal_nominal=1  etaDer_modal_nominal=1
      settings: InternalSimscapePortConfiguration="{\"Bottom\":[],\"Left\":[{\"id\":\"B\",\"label\":\"B\",\"type\":\"foundation.mechanical.rotational.rotational\"}],\"Right\":[{\"id\":\"F\",\"label\":\"F\",\"type\":\"foundation.mechanical.rotational.rotational\"}],\"Top\":[]}"
  Flexible Shaft4 : sdl_lib/Couplings & Drives/Flexible Shaft  modelTorsion=true  modelTransverse=false  n_segments=1  parameterization=sdl.enum.shaftParameterization.StiffnessInertia  length=1 m  lengths=[1, .5, .25] m  shaft_stiffness=2e5 N*m/rad  shaft_inertia=0.02 kg*m^2  shaft_stiffnesses=[400000, 200000, 100000] N*m/rad  shaft_inertias=[.025, .02, .015] kg*m^2  eiIN=5e5 Pa*m^4  rhoaIN=19 kg/m  eiINs=[600000, 500000, 400000] Pa*m^4  rhoaINs=[20, 19, 18] kg/m  density=7.8e3 kg/m^3  shear_modulus=7.93e9 Pa  elastic_modulus=200e9 Pa  shaft_construction=sdl.enum.shaftConstruction.solid  diameter_outer=0.075 m  diameter_inner=0.05 m  diameter_outers=[.085, .075, .065] m  diameter_inners=[.055, .05, .045] m  damping_ratio=0.01  mu_visc_BF=[0, 0] N*m*s/rad  mu_visc=[0, 0] N*m*s/rad  initial_deflection=0 rad  initial_velocity=0 rpm  num_supports=sdl.enum.num_supports.two  z_support=[0, 1] m  boundaryB1=sdl.enum.shaftSupport.clamp  DrotB1_row=[1000, 1000] N*m*s/rad  DtransB1_row=[20000, -44000, -44000, 350000] N*s/m  DtransB1_w_mat=[20000, -44000, -44000, 350000; 10000, -25000, -25000, 140000; 5000, -10000, -10000, 20000] N*s/m  KrotB1_row=[10000, 10000] N*m/rad  KtransB1_row=[1000000, -200000, -300000, 5000000] N/m  KtransB1_w_mat=[1000000, -600000, -3500000, 8000000; 1000000, -200000, -3000000, 5000000; 1000000, -50000, -2500000, 3000000] N/m  boundaryI1=sdl.enum.shaftSupport.clamp  DrotI1_row=[1000, 1000] N*m*s/rad  DtransI1_row=[20000, -44000, -44000, 350000] N*s/m  DtransI1_w_mat=[20000, -44000, -44000, 350000; 10000, -25000, -25000, 140000; 5000, -10000, -10000, 20000] N*s/m  KrotI1_row=[10000, 10000] N*m/rad  KtransI1_row=[1000000, -200000, -300000, 5000000] N/m  KtransI1_w_mat=[1000000, -600000, -3500000, 8000000; 1000000, -200000, -3000000, 5000000; 1000000, -50000, -2500000, 3000000] N/m  boundaryI2=sdl.enum.shaftSupport.clamp  DrotI2_row=[1000, 1000] N*m*s/rad  DtransI2_row=[20000, -44000, -44000, 350000] N*s/m  DtransI2_w_mat=[20000, -44000, -44000, 350000; 10000, -25000, -25000, 140000; 5000, -10000, -10000, 20000] N*s/m  KrotI2_row=[10000, 10000] N*m/rad  KtransI2_row=[1000000, -200000, -300000, 5000000] N/m  KtransI2_w_mat=[1000000, -600000, -3500000, 8000000; 1000000, -200000, -3000000, 5000000; 1000000, -50000, -2500000, 3000000] N/m  boundaryF1=sdl.enum.shaftSupport.clamp  DrotF1_row=[1000, 1000] N*m*s/rad  DtransF1_row=[20000, -44000, -44000, 350000] N*s/m  DtransF1_w_mat=[20000, -44000, -44000, 350000; 10000, -25000, -25000, 140000; 5000, -10000, -10000, 20000] N*s/m  KrotF1_row=[10000, 10000] N*m/rad  KtransF1_row=[1000000, -200000, -300000, 5000000] N/m  KtransF1_w_mat=[1000000, -600000, -3500000, 8000000; 1000000, -200000, -3000000, 5000000; 1000000, -50000, -2500000, 3000000] N/m  bearing_speed=[200, 500, 1500] rpm  alpha=10 1/s  beta=1e-8 s  noDisk=sdl.enum.shaftDisks.none  zDisk=0.5 m  mDiskIN=2 kg  IdDiskIN=0.025 kg*m^2  IpDiskIN=0.050 kg*m^2  enable_static_unbalance=true  offsetMR=[.01, .01] kg*m  offsetMR_initialAngleIN=[0, pi] rad  offsetMassLocation=[.33, .67] m  enable_external_force=false  externalForce=[1, 2] N  externalForceHarmonic=[.5, 2]  externalLoadAngle=[pi / 2, 3 * pi / 4] rad  zExternalLoad=[.25, .75] m  AnalysisMethod=sdl.enum.bendingAnalysisMethod.LumpedMass  ModeInputMethod=sdl.enum.modeInputMethod.SimscapeDetermined  numModesIn=6  mode_speed_dependency=sdl.enum.mode_speed_dependency.Static  OmegaNom=5000 rpm  wMax=1e8 rpm  dz=0.01 m  userMode_w=[280, 644, 615, 1285] rad/s  userMode_w_mat=[257, 780, 580, 1560; 280, 644, 615, 1285; 294, 513, 636, 1020] rad/s  userMode_z=[0, .1, .2, .3, .4, .5, .6, .7, .8, .9, 1] m  userMode_shapeX=[.1648, .0086, -.2759, .0162; .1671, .0093, -.2231, .0133; .1691, .01, -.1689, .0102; .1707, .0105, -.1135, .007; .1717, .0108, -.057, .0035; .1721, .0109, 0, 0; .1717, .0108, .057, -.0035; .1707, .0105, .1135, -.007; .1691, .01, .1689, -.0102; .1671, .0093, .2231, -.0133; .1648, .0086, .2759, -.0162]  userMode_shapeX_mat=cat(3, [.1842, .0134, -.3072, .0272; .1863, .0152, -.2482, .0226; .1882, .0169, -.1878, .0176; .1897, .0182, -.1261, .0121; .1906, .019, -.0634, .0062; .191, .0193, 0, 0; .1906, .019, .0634, -.0062; .1897, .0182, .1261, -.0121; .1882, .0169, .1878, -.0176; .1863, .0152, .2482, -.0226; .1842, .0134, .3072, -.0272], [.1648, .0086, -.2759, .0162; .1671, .0093, -.2231, .0133; .1691, .01, -.1689, .0102; .1707, .0105, -.1135, .007; .1717, .0108, -.057, .0035; .1721, .0109, 0, 0; .1717, .0108, .057, -.0035; .1707, .0105, .1135, -.007; .1691, .01, .1689, -.0102; .1671, .0093, .2231, -.0133; .1648, .0086, .2759, -.0162], [.1291, .0046, -.2166, .0082; .131, .0048, -.1751, .0067; .1327, .005, -.1327, .0051; .1341, .0052, -.0891, .0035; .135, .0053, -.0448, .0017; .1353, .0053, 0, 0; .135, .0053, .0448, -.0017; .1341, .0052, .0891, -.0035; .1327, .005, .1327, -.0051; .131, .0048, .1751, -.0067; .1291, .0046, .2166, -.0082])  userMode_shapeY=[.1193, -.1784, -.1997, -.3348; .1209, -.1933, -.1615, -.2751; .1224, -.2068, -.1223, -.2119; .1235, -.2176, -.0821, -.1445; .1243, -.2245, -.0413, -.0734; .1246, -.2269, 0, 0; .1243, -.2245, .0413, .0734; .1235, -.2176, .0821, .1445; .1224, -.2068, .1223, .2119; .1209, -.1933, .1615, .2751; .1193, -.1784, .1997, .3348]  userMode_shapeY_mat=cat(3, [.0885, -.1625, -.1475, -.3301; .0895, -.1847, -.1192, -.2745; .0904, -.2048, -.0902, -.2141; .0911, -.2209, -.0606, -.1475; .0916, -.2313, -.0304, -.0754; .0917, -.2349, 0, 0; .0916, -.2313, .0304, .0754; .0911, -.2209, .0606, .1475; .0904, -.2048, .0902, .2141; .0895, -.1847, .1192, .2745; .0885, -.1625, .1475, .3301], [.1193, -.1784, -.1997, -.3348; .1209, -.1933, -.1615, -.2751; .1224, -.2068, -.1223, -.2119; .1235, -.2176, -.0821, -.1445; .1243, -.2245, -.0413, -.0734; .1246, -.2269, 0, 0; .1243, -.2245, .0413, .0734; .1235, -.2176, .0821, .1445; .1224, -.2068, .1223, .2119; .1209, -.1933, .1615, .2751; .1193, -.1784, .1997, .3348], [.1566, -.1901, -.2628, -.3377; .1589, -.1994, -.2125, -.2753; .161, -.2079, -.1609, -.2103; .1627, -.2146, -.1081, -.1424; .1638, -.219, -.0544, -.0719; .1642, -.2205, 0, 0; .1638, -.219, .0544, .0719; .1627, -.2146, .1081, .1424; .161, -.2079, .1609, .2103; .1589, -.1994, .2125, .2753; .1566, -.1901, .2628, .3377])  eta_lumped_nominal=1  etaDer_lumped_nominal=1  eta_modal_nominal=1  etaDer_modal_nominal=1
      settings: InternalSimscapePortConfiguration="{\"Bottom\":[],\"Left\":[{\"id\":\"B\",\"label\":\"B\",\"type\":\"foundation.mechanical.rotational.rotational\"}],\"Right\":[{\"id\":\"F\",\"label\":\"F\",\"type\":\"foundation.mechanical.rotational.rotational\"}],\"Top\":[]}"
  Ideal Torque Sensor1 : fl_lib/Mechanical/Mechanical Sensors/Ideal Torque Sensor
  Ideal Torque Sensor2 : fl_lib/Mechanical/Mechanical Sensors/Ideal Torque Sensor
  Mechanical Rotational Reference1 : fl_lib/Mechanical/Rotational Elements/Mechanical Rotational Reference
  Mechanical Rotational Reference2 : fl_lib/Mechanical/Rotational Elements/Mechanical Rotational Reference
  Motor Pinion Ratio : sdl_lib/Gears/Simple Gear  ratio=motorToCSGearRatio  rotation_direction=sdl.enum.shaftOutputDirection.opposite  friction_model=sdl.enum.gear_efficiencies_load.off  T_noload=0.1 N*m  T_nom=5 N*m  efficiency_nom=0.8  efficiency=0.8  temperature_TLU=[280, 300, 320] K  load_TLU=[1, 5, 10] N*m  efficiency_TLU=[.95, .9, .85]  efficiency_TLU2=[.85, .8, .75; .95, .9, .85; .85, .8, .7]  w_thr=0.01 rad/s  pwr_thr=0.001 W  enable_backlash=true  hardstop_model=simscape.enum.hardstop.smooth  backlash_distance=flexDLParams.gearBox.gear1BackLash mm  r_base=flexDLParams.gearBox.gear1BaseRadius m  transition=1e-4 mm  backlash_stiffness=flexDLParams.gearBox.gear1Stiffness N/m  backlash_damping=flexDLParams.gearBox.gear1Damping N*s/m  coeff_rest=0.7  v_tol=0.001 m/s  f_tol=0.001 N  mu_visc=flexDLParams.gearBox.gear2ViscousDampingCoefficients N*m*s/rad  thermal_mass=50 J/K  temperature_specify=off  temperature_priority=High  temperature=300 K  temperature_nominal_specify=off  temperature_nominal_value=1  temperature_nominal_unit=K  x_backlash_specify=off  x_backlash_priority=None  x_backlash=0 mm  x_backlash_nominal_specify=off  x_backlash_nominal_value=1  x_backlash_nominal_unit=mm  f_hardstop_specify=off  f_hardstop_priority=None  f_hardstop=0 N  f_hardstop_nominal_specify=off  f_hardstop_nominal_value=1  f_hardstop_nominal_unit=N  v_backlash_specify=off  v_backlash_priority=None  v_backlash=0 m/s  v_backlash_nominal_specify=off  v_backlash_nominal_value=1  v_backlash_nominal_unit=m/s
  TRQ2RadialLoad1 : Subsystem
  TRQ2RadialLoad2 : Subsystem
  out : PMIOPort  Side=Left
  O : PMIOPort  Port=2  Side=Right
  connections:
  TRQ2RadialLoad1/RConn1 -- Bearing3/LConn2
  Ideal Torque Sensor2/RConn1 -- Bearing3/RConn1
  Ideal Torque Sensor2/LConn1 -- Flexible Shaft2/RConn1
  Ideal Torque Sensor2/RConn2 -- TRQ2RadialLoad1/LConn1
  TRQ2RadialLoad2/RConn1 -- Bearing4/LConn2
  Ideal Torque Sensor1/LConn1 -- Motor Pinion Ratio/RConn1
  Ideal Torque Sensor1/RConn1 -- Bearing4/RConn1
  Ideal Torque Sensor1/RConn2 -- TRQ2RadialLoad2/LConn1
  Flexible Shaft2/LConn1 -- Counter Shaft Ratio/RConn1
  Counter Shaft Ratio/LConn1 -- Flexible Shaft4/RConn1 -- CS Gear-2/LConn1
  Motor Pinion Ratio/LConn1 -- O/RConn1
  Mechanical Rotational Reference2/LConn1 -- Bearing3/RConn2
  Mechanical Rotational Reference1/LConn1 -- Bearing4/RConn2
  Bearing3/LConn1 -- out/RConn1
  Bearing4/LConn1 -- Flexible Shaft3/LConn1
  CS Gear1/LConn1 -- Flexible Shaft3/RConn1 -- Flexible Shaft4/LConn1

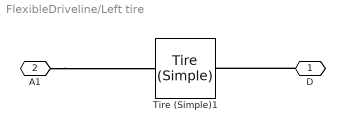
== system FlexibleDriveline/Left tire ==
  Tire (Simple)1 : sdl_lib/Tires & Vehicles/Tire (Simple)  r_tire=flexDLParams.gearBox.tireR m  model_compliance=sdl.enum.compliance.on  stiffness=1e6 N/m  damping=1000 N*s/m  model_inertia=sdl.enum.model_inertia.on  tire_inertia=1 kg*m^2  initial_velocity=0 rad/s
      settings: InternalSimscapePortConfiguration="{\"Bottom\":[],\"Left\":[{\"id\":\"A\",\"label\":\"A\",\"type\":\"foundation.mechanical.rotational.rotational\"}],\"Right\":[{\"id\":\"H\",\"label\":\"H\",\"type\":\"foundation.mechanical.translational.translational\"}],\"Top\":[]}"
  D : PMIOPort  Side=Right
  A1 : PMIOPort  Port=2  Side=Right
  connections:
  A1/RConn1 -- Tire (Simple)1/LConn1
  D/RConn1 -- Tire (Simple)1/RConn1
